simulink model "smart_library"  (R2026b)
settings: Solver=VariableStepAuto  StopTime=660
libraries: simulink x4
settings Model: Creator=sarag  LastModifiedBy=sarag

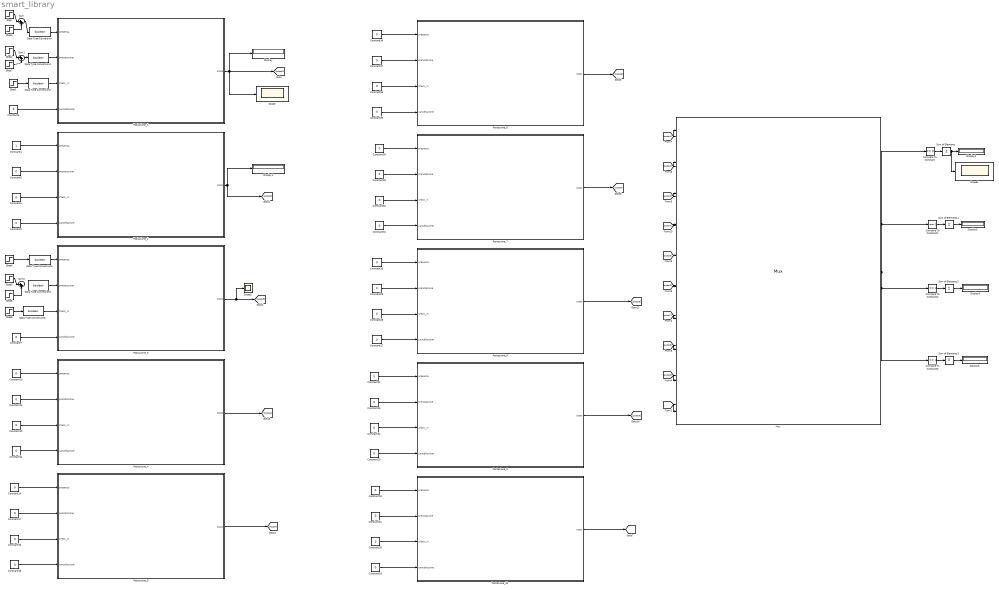
== system smart_library ==
  Compare To Constant : simulink/Logic and Bit Operations/Compare To Constant  relop===  const=0  OutDataTypeStr=boolean
  Compare To Constant1 : simulink/Logic and Bit Operations/Compare To Constant  relop===  const=1  OutDataTypeStr=boolean
  Compare To Constant2 : simulink/Logic and Bit Operations/Compare To Constant  relop===  const=2  OutDataTypeStr=boolean
  Compare To Constant3 : simulink/Logic and Bit Operations/Compare To Constant  relop===  const=3  OutDataTypeStr=boolean
  Constant1 : Constant  OutDataTypeStr=boolean
  Constant{2..5,7,10..37} (33 alike) : Constant  Value=0  OutDataTypeStr=boolean
  Data Type Conversion{,1..5} (6 alike) : DataTypeConversion  OutDataTypeStr=boolean  SaturateOnIntegerOverflow=off  RndMeth=Floor
  Display{,1..5} (6 alike) : Display
  Mux : Mux  Inputs=10
  Postazione_1 : Stateflow chart  TreatAsAtomicUnit=on
  Postazione_10 : Stateflow chart  TreatAsAtomicUnit=on
  Postazione_2 : Stateflow chart  TreatAsAtomicUnit=on
  Postazione_3 : Stateflow chart  TreatAsAtomicUnit=on
  Postazione_4 : Stateflow chart  TreatAsAtomicUnit=on
  Postazione_5 : Stateflow chart  TreatAsAtomicUnit=on
  Postazione_6 : Stateflow chart  TreatAsAtomicUnit=on
  Postazione_7 : Stateflow chart  TreatAsAtomicUnit=on
  Postazione_8 : Stateflow chart  TreatAsAtomicUnit=on
  Postazione_9 : Stateflow chart  TreatAsAtomicUnit=on
  Scope : Scope
      settings: ActiveDisplayYMinimum=-0.37499999999999989  ActiveDisplayYMaximum=3.375
  Scope1 : Scope
      settings: ActiveDisplayYMinimum=0.740548065650645  ActiveDisplayYMaximum=10.375
  Scope2 : Scope
      settings: ActiveDisplayYMinimum=-0.37499999999999989  ActiveDisplayYMaximum=3.375  DataLoggingVariableName=ScopeData2
  Step : Step  Time=20  SampleTime=0
  Step1 : Step  Time=20  SampleTime=0
  Step2 : Step  Time=5  SampleTime=0
  Step3 : Step  Time=40  FinalValue=-1  SampleTime=0
  Step4 : Step  Time=30  SampleTime=0
  Step5 : Step  Time=10  SampleTime=0
  Step6 : Step  Time=11  FinalValue=-1  SampleTime=0
  Step7 : Step  Time=6  FinalValue=-1  SampleTime=0
  Step8 : Step  Time=30  SampleTime=0
  Sum : Sum  Inputs=|++
  Sum of Elements{,1..3} (4 alike) : Sum  Inputs=+
  Sum1 : Sum  Inputs=|++
  Sum2 : Sum  Inputs=|++
  wires:
  Step1/1 -> Data Type Conversion2/1
  Constant3/1 -> Postazione_1/4(cancellazione)
  Postazione_1/1(stato) -> [posto1], Scope/1, Display/1
  Data Type Conversion/1 -> Postazione_1/1(presenza)
  Data Type Conversion2/1 -> Postazione_1/3(check_in)
  Data Type Conversion1/1 -> Postazione_1/2(prenotazione)
  Step3/1 -> Sum/2
  Step/1 -> Sum/1
  Sum/1 -> Data Type Conversion/1
  Postazione_2/1(stato) -> [posto2], Display1/1
  Constant1/1 -> Postazione_2/1(presenza)
  Constant5/1 -> Postazione_2/2(prenotazione)
  Constant4/1 -> Postazione_2/3(check_in)
  Constant2/1 -> Postazione_2/4(cancellazione)
  Constant7/1 -> Postazione_3/4(cancellazione)
  Constant11/1 -> Postazione_4/4(cancellazione)
  Constant13/1 -> Postazione_4/2(prenotazione)
  Constant12/1 -> Postazione_4/3(check_in)
  Constant10/1 -> Postazione_4/1(presenza)
  Constant15/1 -> Postazione_5/4(cancellazione)
  Constant17/1 -> Postazione_5/2(prenotazione)
  Constant16/1 -> Postazione_5/3(check_in)
  Constant14/1 -> Postazione_5/1(presenza)
  Constant19/1 -> Postazione_10/4(cancellazione)
  Constant21/1 -> Postazione_10/2(prenotazione)
  Constant20/1 -> Postazione_10/3(check_in)
  Constant18/1 -> Postazione_10/1(presenza)
  Constant23/1 -> Postazione_9/4(cancellazione)
  Constant25/1 -> Postazione_9/2(prenotazione)
  Constant24/1 -> Postazione_9/3(check_in)
  Constant22/1 -> Postazione_9/1(presenza)
  Constant27/1 -> Postazione_8/4(cancellazione)
  Constant29/1 -> Postazione_8/2(prenotazione)
  Constant28/1 -> Postazione_8/3(check_in)
  Constant26/1 -> Postazione_8/1(presenza)
  Constant31/1 -> Postazione_7/4(cancellazione)
  Constant33/1 -> Postazione_7/2(prenotazione)
  Constant32/1 -> Postazione_7/3(check_in)
  Constant30/1 -> Postazione_7/1(presenza)
  Constant35/1 -> Postazione_6/4(cancellazione)
  Constant37/1 -> Postazione_6/2(prenotazione)
  Constant36/1 -> Postazione_6/3(check_in)
  Constant34/1 -> Postazione_6/1(presenza)
  Postazione_3/1(stato) -> Scope2/1, [posto3]
  Postazione_4/1(stato) -> [posto4]
  Postazione_5/1(stato) -> [posto5]
  Postazione_6/1(stato) -> [posto6]
  Postazione_7/1(stato) -> [posto7]
  Postazione_8/1(stato) -> [posto8]
  Postazione_9/1(stato) -> [posto9]
  Postazione_10/1(stato) -> [posto10]
  [posto10] -> Mux/10
  [posto1] -> Mux/1
  [posto2] -> Mux/2
  [posto3] -> Mux/3
  [posto9] -> Mux/9
  [posto8] -> Mux/8
  [posto7] -> Mux/7
  [posto4] -> Mux/4
  [posto5] -> Mux/5
  [posto6] -> Mux/6
  Compare To Constant/1 -> Sum of Elements/1
  Sum of Elements/1 -> Scope1/1, Display2/1
  Sum of Elements1/1 -> Display3/1
  Compare To Constant1/1 -> Sum of Elements1/1
  Compare To Constant2/1 -> Sum of Elements2/1
  Sum of Elements2/1 -> Display4/1
  Mux/1 -> Compare To Constant2/1, Compare To Constant3/1, Compare To Constant/1, Compare To Constant1/1
  Sum of Elements3/1 -> Display5/1
  Compare To Constant3/1 -> Sum of Elements3/1
  Data Type Conversion3/1 -> Postazione_3/2(prenotazione)
  Step7/1 -> Sum1/2
  Sum1/1 -> Data Type Conversion1/1
  Step2/1 -> Sum1/1
  Data Type Conversion4/1 -> Postazione_3/1(presenza)
  Step4/1 -> Data Type Conversion4/1
  Step5/1 -> Sum2/1
  Step6/1 -> Sum2/2
  Step8/1 -> Data Type Conversion5/1
  Data Type Conversion5/1 -> Postazione_3/3(check_in)

== stateflow chart smart_library/Postazione_5 ==
  state LIBERO
    entry: stato = 0;
  state PRENOTATO
    entry: stato = 1;
  state OCCUPATO
    entry: stato = 2;
  state ASSENTE
    entry: stato = 3;
  (default) -> LIBERO
  LIBERO -> PRENOTATO [order 1] : [prenotazione == 1]
  PRENOTATO -> LIBERO [order 2] : [cancellazione == 1]
  PRENOTATO -> LIBERO [order 3] : [after(900,sec)]
  PRENOTATO -> OCCUPATO [order 1] : [presenza == 1 && check_in == 1]
  LIBERO -> OCCUPATO [order 2] : [presenza == 1 && prenotazione == 0]
  ASSENTE -> LIBERO [order 2] : [after(600,sec) && presenza == 0]
  OCCUPATO -> ASSENTE : [presenza == 0]
  ASSENTE -> OCCUPATO [order 1] : [presenza == 1]
  data: stato output; presenza input boolean size=1; prenotazione input boolean size=1; check_in input boolean size=1; cancellazione input boolean size=1

== stateflow chart smart_library/Postazione_6 ==
  state LIBERO
    entry: stato = 0;
  state PRENOTATO
    entry: stato = 1;
  state OCCUPATO
    entry: stato = 2;
  state ASSENTE
    entry: stato = 3;
  (default) -> LIBERO
  LIBERO -> PRENOTATO [order 1] : [prenotazione == 1]
  PRENOTATO -> LIBERO [order 2] : [cancellazione == 1]
  PRENOTATO -> LIBERO [order 3] : [after(900,sec)]
  PRENOTATO -> OCCUPATO [order 1] : [presenza == 1 && check_in == 1]
  LIBERO -> OCCUPATO [order 2] : [presenza == 1 && prenotazione == 0]
  ASSENTE -> LIBERO [order 2] : [after(600,sec) && presenza == 0]
  OCCUPATO -> ASSENTE : [presenza == 0]
  ASSENTE -> OCCUPATO [order 1] : [presenza == 1]
  data: stato output; presenza input boolean size=1; prenotazione input boolean size=1; check_in input boolean size=1; cancellazione input boolean size=1

== stateflow chart smart_library/Postazione_7 ==
  state LIBERO
    entry: stato = 0;
  state PRENOTATO
    entry: stato = 1;
  state OCCUPATO
    entry: stato = 2;
  state ASSENTE
    entry: stato = 3;
  (default) -> LIBERO
  LIBERO -> PRENOTATO [order 1] : [prenotazione == 1]
  PRENOTATO -> LIBERO [order 2] : [cancellazione == 1]
  PRENOTATO -> LIBERO [order 3] : [after(900,sec)]
  PRENOTATO -> OCCUPATO [order 1] : [presenza == 1 && check_in == 1]
  LIBERO -> OCCUPATO [order 2] : [presenza == 1 && prenotazione == 0]
  ASSENTE -> LIBERO [order 2] : [after(600,sec) && presenza == 0]
  OCCUPATO -> ASSENTE : [presenza == 0]
  ASSENTE -> OCCUPATO [order 1] : [presenza == 1]
  data: stato output; presenza input boolean size=1; prenotazione input boolean size=1; check_in input boolean size=1; cancellazione input boolean size=1

== stateflow chart smart_library/Postazione_8 ==
  state LIBERO
    entry: stato = 0;
  state PRENOTATO
    entry: stato = 1;
  state OCCUPATO
    entry: stato = 2;
  state ASSENTE
    entry: stato = 3;
  (default) -> LIBERO
  LIBERO -> PRENOTATO [order 1] : [prenotazione == 1]
  PRENOTATO -> LIBERO [order 2] : [cancellazione == 1]
  PRENOTATO -> LIBERO [order 3] : [after(900,sec)]
  PRENOTATO -> OCCUPATO [order 1] : [presenza == 1 && check_in == 1]
  LIBERO -> OCCUPATO [order 2] : [presenza == 1 && prenotazione == 0]
  ASSENTE -> LIBERO [order 2] : [after(600,sec) && presenza == 0]
  OCCUPATO -> ASSENTE : [presenza == 0]
  ASSENTE -> OCCUPATO [order 1] : [presenza == 1]
  data: stato output; presenza input boolean size=1; prenotazione input boolean size=1; check_in input boolean size=1; cancellazione input boolean size=1

== stateflow chart smart_library/Postazione_9 ==
  state LIBERO
    entry: stato = 0;
  state PRENOTATO
    entry: stato = 1;
  state OCCUPATO
    entry: stato = 2;
  state ASSENTE
    entry: stato = 3;
  (default) -> LIBERO
  LIBERO -> PRENOTATO [order 1] : [prenotazione == 1]
  PRENOTATO -> LIBERO [order 2] : [cancellazione == 1]
  PRENOTATO -> LIBERO [order 3] : [after(900,sec)]
  PRENOTATO -> OCCUPATO [order 1] : [presenza == 1 && check_in == 1]
  LIBERO -> OCCUPATO [order 2] : [presenza == 1 && prenotazione == 0]
  ASSENTE -> LIBERO [order 2] : [after(600,sec) && presenza == 0]
  OCCUPATO -> ASSENTE : [presenza == 0]
  ASSENTE -> OCCUPATO [order 1] : [presenza == 1]
  data: stato output; presenza input boolean size=1; prenotazione input boolean size=1; check_in input boolean size=1; cancellazione input boolean size=1

== stateflow chart smart_library/Postazione_10 ==
  state LIBERO
    entry: stato = 0;
  state PRENOTATO
    entry: stato = 1;
  state OCCUPATO
    entry: stato = 2;
  state ASSENTE
    entry: stato = 3;
  (default) -> LIBERO
  LIBERO -> PRENOTATO [order 1] : [prenotazione == 1]
  PRENOTATO -> LIBERO [order 2] : [cancellazione == 1]
  PRENOTATO -> LIBERO [order 3] : [after(900,sec)]
  PRENOTATO -> OCCUPATO [order 1] : [presenza == 1 && check_in == 1]
  LIBERO -> OCCUPATO [order 2] : [presenza == 1 && prenotazione == 0]
  ASSENTE -> LIBERO [order 2] : [after(600,sec) && presenza == 0]
  OCCUPATO -> ASSENTE : [presenza == 0]
  ASSENTE -> OCCUPATO [order 1] : [presenza == 1]
  data: stato output; presenza input boolean size=1; prenotazione input boolean size=1; check_in input boolean size=1; cancellazione input boolean size=1

== stateflow chart smart_library/Postazione_2 ==
  state LIBERO
    entry: stato = 0;
  state PRENOTATO
    entry: stato = 1;
  state OCCUPATO
    entry: stato = 2;
  state ASSENTE
    entry: stato = 3;
  (default) -> LIBERO
  LIBERO -> PRENOTATO [order 1] : [prenotazione == 1]
  PRENOTATO -> LIBERO [order 2] : [cancellazione == 1]
  PRENOTATO -> LIBERO [order 3] : [after(900,sec)]
  PRENOTATO -> OCCUPATO [order 1] : [presenza == 1 && check_in == 1]
  LIBERO -> OCCUPATO [order 2] : [presenza == 1 && prenotazione == 0]
  ASSENTE -> LIBERO [order 2] : [after(600,sec) && presenza == 0]
  OCCUPATO -> ASSENTE : [presenza == 0]
  ASSENTE -> OCCUPATO [order 1] : [presenza == 1]
  data: stato output; presenza input boolean size=1; prenotazione input boolean size=1; check_in input boolean size=1; cancellazione input boolean size=1

== stateflow chart smart_library/Postazione_3 ==
  state LIBERO
    entry: stato = 0;
  state PRENOTATO
    entry: stato = 1;
  state OCCUPATO
    entry: stato = 2;
  state ASSENTE
    entry: stato = 3;
  (default) -> LIBERO
  LIBERO -> PRENOTATO [order 1] : [prenotazione == 1]
  PRENOTATO -> LIBERO [order 2] : [cancellazione == 1]
  PRENOTATO -> LIBERO [order 3] : [after(900,sec)]
  PRENOTATO -> OCCUPATO [order 1] : [presenza == 1 && check_in == 1]
  LIBERO -> OCCUPATO [order 2] : [presenza == 1 && prenotazione == 0]
  ASSENTE -> LIBERO [order 2] : [after(600,sec) && presenza == 0]
  OCCUPATO -> ASSENTE : [presenza == 0]
  ASSENTE -> OCCUPATO [order 1] : [presenza == 1]
  data: stato output; presenza input boolean size=1; prenotazione input boolean size=1; check_in input boolean size=1; cancellazione input boolean size=1

== stateflow chart smart_library/Postazione_1 ==
  state LIBERO
    entry: stato = 0;
  state PRENOTATO
    entry: stato = 1;
  state OCCUPATO
    entry: stato = 2;
  state ASSENTE
    entry: stato = 3;
  (default) -> LIBERO
  LIBERO -> PRENOTATO [order 1] : [prenotazione == 1]
  PRENOTATO -> LIBERO [order 2] : [cancellazione == 1]
  PRENOTATO -> LIBERO [order 3] : [after(900,sec)]
  PRENOTATO -> OCCUPATO [order 1] : [presenza == 1 && check_in == 1]
  LIBERO -> OCCUPATO [order 2] : [presenza == 1 && prenotazione == 0]
  ASSENTE -> LIBERO [order 2] : [after(600,sec) && presenza == 0]
  OCCUPATO -> ASSENTE : [presenza == 0]
  ASSENTE -> OCCUPATO [order 1] : [presenza == 1]
  data: stato output; presenza input boolean size=1; prenotazione input boolean size=1; check_in input boolean size=1; cancellazione input boolean size=1

== stateflow chart smart_library/Postazione_4 ==
  state LIBERO
    entry: stato = 0;
  state PRENOTATO
    entry: stato = 1;
  state OCCUPATO
    entry: stato = 2;
  state ASSENTE
    entry: stato = 3;
  (default) -> LIBERO
  LIBERO -> PRENOTATO [order 1] : [prenotazione == 1]
  PRENOTATO -> LIBERO [order 2] : [cancellazione == 1]
  PRENOTATO -> LIBERO [order 3] : [after(900,sec)]
  PRENOTATO -> OCCUPATO [order 1] : [presenza == 1 && check_in == 1]
  LIBERO -> OCCUPATO [order 2] : [presenza == 1 && prenotazione == 0]
  ASSENTE -> LIBERO [order 2] : [after(600,sec) && presenza == 0]
  OCCUPATO -> ASSENTE : [presenza == 0]
  ASSENTE -> OCCUPATO [order 1] : [presenza == 1]
  data: stato output; presenza input boolean size=1; prenotazione input boolean size=1; check_in input boolean size=1; cancellazione input boolean size=1
